simulink model "mod_fsk2"  (R2024b)
settings: Solver=FixedStepDiscrete  StartTime=0.0  StopTime=1  FixedStep=3.1250000000000001e-05  RelTol=1e-3
model workspace (MAT data in the model file):
  M = 2
  Ts = 0.001
  decalage = 0.00096875
  df_ol = 1
  excursion = 1000
  fc = 4000
  fs = 32000
  graine = 7
  h_pb = [-0.000256045267055 0.000136691402229 0.000538557567029 0.00083782800937 0.000906112776054 0.000635343207351 -9.88408387428e-19 -0.000882285176312 -0.00173231428985 -0.00216653683552 -0.00183353726722 -0.000591229449117 0.00134908111707 0.00339366489502 0.00470388827103 0.00448811530924 0.00236098666957 -0.00137079710138 -0.00564080523999 -0.00885900199847 -0.00942825317846 -0.00639498356516 4.76480364404e-18 0.00811457160728 0.0152007196615 0.0181972737526 0.0148244343916 0.00463627974173 -0.0103566731882 -0.0257918928366 -0.0358732474797 -0.0349225637276 -0.0191464255819 0.0119199755455 0.0547815288845 0.102439365205 0.145889082105 0.176289643262 0.187206897605 0.176289643262 0.145889082105 0.102439365205 0.0547815288845 0.0119199755455 -0.0191464255819 -0.0349225637276 -0.0358732474797 -0.0257918928366 -0.0103566731882 0.00463627974173 0.0148244343916 0.0181972737526 0.0152007196615 0.00811457160728 4.76480364404e-18 -0.00639498356516 -0.00942825317846 -0.00885900199847 -0.00564080523999 -0.00137079710138 0.00236098666957 0.00448811530924 0.00470388827103 0.00339366489502 0.00134908111707 -0.000591229449117 -0.00183353726722 -0.00216653683552 -0.00173231428985 -0.000882285176312 -9.88408387428e-19 0.000635343207351 0.000906112776054 0.00083782800937 0.000538557567029 0.000136691402229 -0.000256045267055]
  h_rx = [0.03125 0.03125 0.03125 0.03125 0.03125 0.03125 0.03125 0.03125 0.03125 0.03125 0.03125 0.03125 0.03125 0.03125 0.03125 0.03125 0.03125 0.03125 0.03125 0.03125 0.03125 0.03125 0.03125 0.03125 0.03125 0.03125 0.03125 0.03125 0.03125 0.03125 0.03125 0.03125]
  ordre = 1
  phi_ol = 0.7
  points = [-1 1]
  ptsI = [-1 1]
  ptsQ = [0 0]
  sigma2 = 0
  sps = 32
undefined symbols (not defined in the file): DiscIntNeverNeededParam
libraries: simulink x2
settings Model: Creator=runner  LastModifiedBy=runner

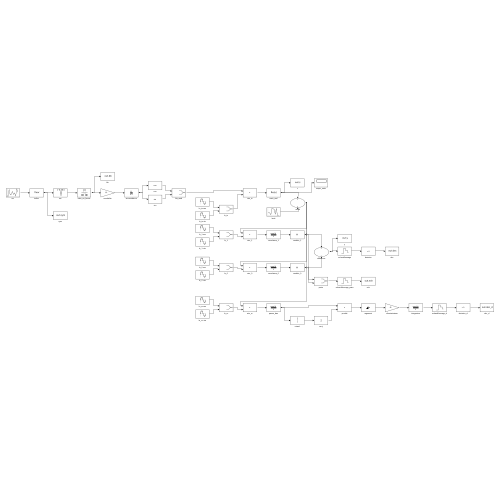
[thumbnail: Simulink's stored preview of the top-level diagram]
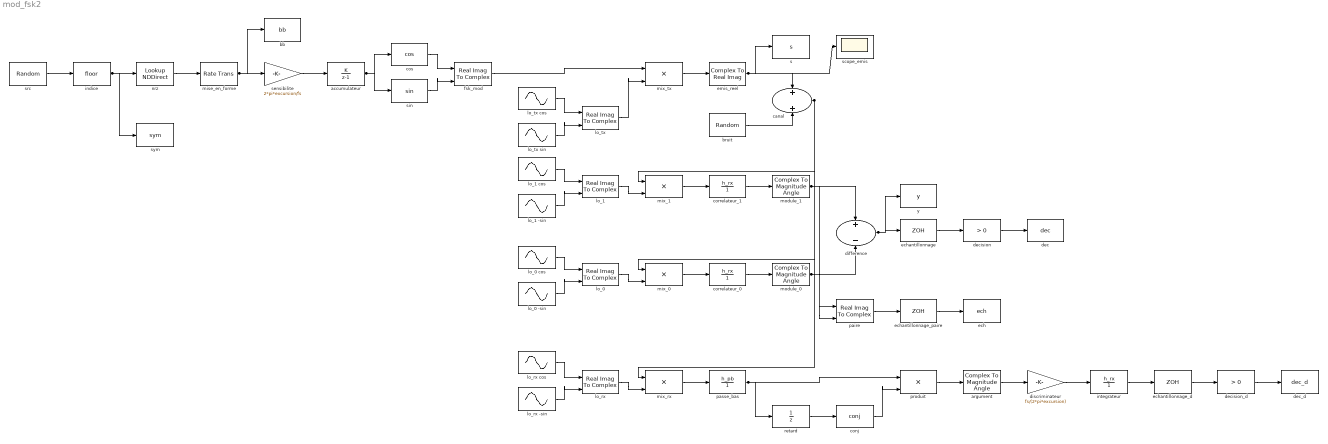
== system mod_fsk2 ==
  accumulateur : DiscreteIntegrator  IntegratorMethod=Accumulation: Forward Euler  SampleTime=1/fs  ICPrevOutput=DiscIntNeverNeededParam  ICPrevScaledInput=DiscIntNeverNeededParam
  argument : ComplexToMagnitudeAngle  Output=Angle
  bb : ToWorkspace  VariableName=bb  SampleTime=-1
  bruit : RandomNumber  Variance=sigma2  Seed=1  SampleTime=1/fs
  canal : Sum
  conj : Math  Operator=conj
  correlateur_0 : DiscreteFilter  Numerator=h_rx  Denominator=1
  correlateur_1 : DiscreteFilter  Numerator=h_rx  Denominator=1
  cos : Trigonometry  Operator=cos
  dec : ToWorkspace  VariableName=dec  SampleTime=-1
  dec_d : ToWorkspace  VariableName=dec_d  SampleTime=-1
  decision : simulink/Logic and Bit Operations/Compare To Zero  relop=>  OutDataTypeStr=boolean
  decision_d : simulink/Logic and Bit Operations/Compare To Zero  relop=>  OutDataTypeStr=boolean
  difference : Sum  Inputs=+-
  discriminateur : Gain  Gain=fs/(2*pi*excursion)
  ech : ToWorkspace  VariableName=ech  SampleTime=-1
  echantillonnage : ZeroOrderHold  SampleTime=[Ts, decalage]
  echantillonnage_d : ZeroOrderHold  SampleTime=[Ts, decalage]
  echantillonnage_paire : ZeroOrderHold  SampleTime=[Ts, decalage]
  emis_reel : ComplexToRealImag  Output=Real
  fsk_mod : RealImagToComplex
  indice : Rounding
  integrateur : DiscreteFilter  Numerator=h_rx  Denominator=1
  lo_0 : RealImagToComplex
  lo_0 -sin : Sin  Amplitude=-2  Frequency=2*pi*(fc-excursion+df_ol)  Phase=phi_ol  SampleTime=1/fs
  lo_0 cos : Sin  Amplitude=2  Frequency=2*pi*(fc-excursion+df_ol)  Phase=phi_ol+pi/2  SampleTime=1/fs
  lo_1 : RealImagToComplex
  lo_1 -sin : Sin  Amplitude=-2  Frequency=2*pi*(fc+excursion+df_ol)  Phase=phi_ol  SampleTime=1/fs
  lo_1 cos : Sin  Amplitude=2  Frequency=2*pi*(fc+excursion+df_ol)  Phase=phi_ol+pi/2  SampleTime=1/fs
  lo_rx : RealImagToComplex
  lo_rx -sin : Sin  Amplitude=-2  Frequency=2*pi*(fc+df_ol)  Phase=phi_ol  SampleTime=1/fs
  lo_rx cos : Sin  Amplitude=2  Frequency=2*pi*(fc+df_ol)  Phase=phi_ol+pi/2  SampleTime=1/fs
  lo_tx : RealImagToComplex
  lo_tx cos : Sin  Frequency=2*pi*fc  Phase=pi/2  SampleTime=1/fs
  lo_tx sin : Sin  Frequency=2*pi*fc  SampleTime=1/fs
  mise_en_forme : RateTransition  OutPortSampleTime=1/fs
  mix_0 : Product
  mix_1 : Product
  mix_rx : Product
  mix_tx : Product
  module_0 : ComplexToMagnitudeAngle  Output=Magnitude
  module_1 : ComplexToMagnitudeAngle  Output=Magnitude
  nrz : LookupNDDirect  NumberOfTableDimensions=1  Table=ptsI
  paire : RealImagToComplex
  passe_bas : DiscreteFilter  Numerator=h_pb  Denominator=1
  produit : Product
  retard : UnitDelay  SampleTime=1/fs  HasFrameUpgradeWarning=on
  s : ToWorkspace  VariableName=s  SampleTime=-1
  scope_emis : Scope
  sensibilite : Gain  Gain=2*pi*excursion/fs
  sin : Trigonometry
  src : UniformRandomNumber  Minimum=0  Maximum=M  Seed=graine  SampleTime=Ts
  sym : ToWorkspace  VariableName=sym  SampleTime=-1
  y : ToWorkspace  VariableName=y  SampleTime=-1
  wires:
  src/1 -> indice/1
  indice/1 -> nrz/1, sym/1
  nrz/1 -> mise_en_forme/1
  mise_en_forme/1 -> bb/1, sensibilite/1
  sensibilite/1 -> accumulateur/1
  accumulateur/1 -> cos/1, sin/1
  cos/1 -> fsk_mod/1
  sin/1 -> fsk_mod/2
  lo_tx cos/1 -> lo_tx/1
  lo_tx sin/1 -> lo_tx/2
  fsk_mod/1 -> mix_tx/1
  lo_tx/1 -> mix_tx/2
  mix_tx/1 -> emis_reel/1
  emis_reel/1 -> canal/1, s/1, scope_emis/1
  bruit/1 -> canal/2
  lo_1 cos/1 -> lo_1/1
  lo_1 -sin/1 -> lo_1/2
  canal/1 -> mix_1/1, mix_0/1, mix_rx/1
  lo_1/1 -> mix_1/2
  mix_1/1 -> correlateur_1/1
  correlateur_1/1 -> module_1/1
  lo_0 cos/1 -> lo_0/1
  lo_0 -sin/1 -> lo_0/2
  lo_0/1 -> mix_0/2
  mix_0/1 -> correlateur_0/1
  correlateur_0/1 -> module_0/1
  module_1/1 -> difference/1, paire/1
  module_0/1 -> difference/2, paire/2
  difference/1 -> y/1, echantillonnage/1
  echantillonnage/1 -> decision/1
  decision/1 -> dec/1
  paire/1 -> echantillonnage_paire/1
  echantillonnage_paire/1 -> ech/1
  lo_rx cos/1 -> lo_rx/1
  lo_rx -sin/1 -> lo_rx/2
  lo_rx/1 -> mix_rx/2
  mix_rx/1 -> passe_bas/1
  passe_bas/1 -> produit/1, retard/1
  retard/1 -> conj/1
  conj/1 -> produit/2
  produit/1 -> argument/1
  argument/1 -> discriminateur/1
  discriminateur/1 -> integrateur/1
  integrateur/1 -> echantillonnage_d/1
  echantillonnage_d/1 -> decision_d/1
  decision_d/1 -> dec_d/1
